simulink model "Y3Tiltrotor_sim3_INDI"  (R2025a)
settings: Solver=ode4  StartTime=0.0  StopTime=70  FixedStep=uavParam.sampleTime  RelTol=1e-3
PreLoadFcn:
  | filepath  = fileparts(get_param(bdroot, 'FileName'))
  | cd(filepath);
InitFcn:
  | Init_sim_INDI;
values from neighbouring files (symbols this model uses):
  control = struct    [Init_sim_INDI.m]
  env = struct    [InitData.m]
  flightState = struct    [Init_sim_INDI.m]
  FWSpeed0 = 15    [Init_sim_INDI.m]
  k_lpf_p = 50    [Init_sim_INDI.m]
  k_lpf_q = 80    [Init_sim_INDI.m]
  k_lpf_r = 5    [Init_sim_INDI.m]
  k_lpf_u = 10    [Init_sim_INDI.m]
  k_lpf_v = 1    [Init_sim_INDI.m]
  k_lpf_w = 50    [Init_sim_INDI.m]
  k_p = 5    [Init_sim_INDI.m]
  k_q = 20    [Init_sim_INDI.m]
  k_r = 1.5    [Init_sim_INDI.m]
  k_u = 0.5    [Init_sim_INDI.m]
  k_v = 0.5    [Init_sim_INDI.m]
  k_w = 2    [Init_sim_INDI.m]
  uavParam = struct    [InitData.m]
undefined symbols (not defined in the file or in its folder): ControlSampleTime, F, Light, MIL, Newton, Raphson
libraries: slpidlib x28, SignalEditorBlockLib x12, simulink x6, aerolibtransform2 x3, sharedtransform x3, robotcorelib x3, matrix_library x3, aerolibasang x2, aerolibutil x2, aerolibwind2 x2, shared6dof x1, aerolibatmos2 x1
(part 4 of 7)

== system Y3Tiltrotor_sim3_INDI/Subsystem/混控器/固定翼混控/固定翼模态混控 ==
  "FixedwingControlOutput " : Inport
  Action Port : ActionPort  ActionPortLabel=case [ 2 ]:
  Bus Creator : BusCreator  Inputs=2
  Bus Creator1 : BusCreator  Inputs=2
  Bus Selector : BusSelector  OutputSignals=Throttle,Tau_z,dE,dA
  Sum : Sum
  Sum1 : Sum  Inputs=+-
  toMultirotorMixer : Outport
  FixedwingCtrlSurface : Outport  Port=2
  wires:
  "FixedwingControlOutput "/1 -> Bus Selector/1
  Bus Selector/3 -> Sum1/1, Sum/1  "<dE>"
  Bus Selector/4 -> Sum1/2, Sum/2  "<dA>"
  Bus Selector/1 -> Bus Creator/1  "<Throttle>"
  Bus Creator/1 -> toMultirotorMixer/1
  Sum/1 -> Bus Creator1/1  "dA1"
  Sum1/1 -> Bus Creator1/2  "dA2"
  Bus Creator1/1 -> FixedwingCtrlSurface/1
  Bus Selector/2 -> Bus Creator/2  "<Tau_z>"

== system Y3Tiltrotor_sim3_INDI/Subsystem/混控器/固定翼混控/旋翼模态混控 ==
  Action Port : ActionPort  ActionPortLabel=case [ 0 ]:
  Bus Creator1 : BusCreator  Inputs=2
  Constant : Constant  Value=0
  Constant1 : Constant  Value=0
  FixedwingCtrlSurface : Outport
  wires:
  Constant1/1 -> Bus Creator1/2  "dA2"
  Constant/1 -> Bus Creator1/1  "dA1"
  Bus Creator1/1 -> FixedwingCtrlSurface/1

== system Y3Tiltrotor_sim3_INDI/Subsystem/混控器/多旋翼混控/Actuator To Voltage ==
  Motor Commands : Inport
  Bus Creator : BusCreator  Inputs=5
  Bus Selector : BusSelector  OutputSignals=w1,w2,w3,Tilt1,Tilt2
  Gain1 : Gain
  Gain2 : Gain
  Gain3 : Gain  Gain=1/(pi/2)
  Gain4 : Gain
  Gain5 : Gain  Gain=1/(pi/2)
  Gain6 : Gain  Commented=on  Gain=1/(uavParam.motor.RPMMAX/60)
  To PWM : Outport
  wires:
  Motor Commands/1 -> Bus Selector/1
  Bus Selector/1 -> Gain2/1  "<w1>"
  Bus Selector/3 -> Gain1/1  "<w3>"
  Bus Selector/2 -> Gain4/1  "<w2>"
  Bus Selector/4 -> Gain3/1  "<Tilt1>"
  Bus Selector/5 -> Gain5/1  "<Tilt2>"
  Gain2/1 -> Bus Creator/1  "w1"
  Gain4/1 -> Bus Creator/2  "w2"
  Gain1/1 -> Bus Creator/3  "w3"
  Gain3/1 -> Bus Creator/4  "Tilt1"
  Gain5/1 -> Bus Creator/5  "Tilt2"
  Bus Creator/1 -> To PWM/1

== system Y3Tiltrotor_sim3_INDI/Subsystem/混控器/多旋翼混控/固定翼模态混控 ==
  toMultirotorMixer : Inport
  Action Port : ActionPort  ActionPortLabel=case [ 2 ]:
  Bus Creator : BusCreator  Inputs=5
  Bus Selector : BusSelector  OutputSignals=Throttle,Tau_z
  Constant1 : Constant  Value=pi/2
  Constant2 : Constant  Value=0
  Constant7 : Constant  Value=pi/2
  Gain : Gain  Gain=1/2
  Gain1 : Gain  Gain=1/2
  Signed Sqrt : Sqrt
  Signed Sqrt1 : Sqrt
  Sum : Sum
  Sum1 : Sum  Inputs=+-
  MultirotorActuator : Outport
  wires:
  toMultirotorMixer/1 -> Bus Selector/1
  Gain/1 -> Signed Sqrt/1
  Constant1/1 -> Bus Creator/5  "Tilt2"
  Constant7/1 -> Bus Creator/4  "Tilt1"
  Gain1/1 -> Signed Sqrt1/1
  Sum1/1 -> Gain1/1
  Constant2/1 -> Bus Creator/3  "w3"
  Sum/1 -> Gain/1
  Bus Selector/1 -> Sum1/1, Sum/1  "<Throttle>"
  Bus Creator/1 -> MultirotorActuator/1
  Bus Selector/2 -> Sum/2, Sum1/2  "<Tau_z>"
  Signed Sqrt/1 -> Bus Creator/1  "w1"
  Signed Sqrt1/1 -> Bus Creator/2  "w2"

== system Y3Tiltrotor_sim3_INDI/Subsystem/混控器/多旋翼混控/旋翼模态混控 ==
  "MultirotorControlOutput " : Inport
  In Bus Element : Inport  Port=2  PortName=states  Element=Euler
  Action Port : ActionPort  ActionPortLabel=case [ 0 ]:
  Bus Creator : BusCreator  Inputs=5
  Bus Selector : BusSelector  Commented=on  OutputSignals=u_z,u_phi,u_theta
  Bus Selector1 : BusSelector  Commented=on  OutputSignals=u_x,u_psi
  Bus Selector2 : BusSelector  OutputSignals=u_z,u_phi,u_theta,u_psi,u_x
  Gain1 : Gain  Commented=on  Gain=1/(cos(asin((uavParam.motor.CQ*uavParam.geom.PropRadius)/(uavParam.motor.CT*0.24))))
  MATLAB Function : MATLAB Function  Commented=on  TreatAsAtomicUnit=on
  MATLAB Function1 : MATLAB Function  Commented=on  TreatAsAtomicUnit=on
  Multirotor Mixer1 : MATLAB Function  Commented=on  TreatAsAtomicUnit=on
  Multirotor Mixer2 (加上重力分量) : MATLAB Function  TreatAsAtomicUnit=on
  Multirotor Mixer3 : MATLAB Function  Commented=on  TreatAsAtomicUnit=on
  Multirotor Mixer4 (对应论文) : MATLAB Function  Commented=on  TreatAsAtomicUnit=on
  Saturation1 : Saturate  UpperLimit=1  LowerLimit=0
  Saturation2 : Saturate  UpperLimit=1  LowerLimit=0
  Saturation3 : Saturate  UpperLimit=1  LowerLimit=0
  Saturation4 : Saturate  UpperLimit=control.maxTiltMR  LowerLimit=control.minTiltMR
  Saturation5 : Saturate  UpperLimit=control.maxTiltMR  LowerLimit=control.minTiltMR
  Selector6 : Selector  InputPortWidth=3  IndexOptions=Index vector (dialog)  Indices=1  OutputSizes=1
  Selector7 : Selector  InputPortWidth=3  IndexOptions=Index vector (dialog)  Indices=2  OutputSizes=1
  Signed Sqrt : Sqrt
  Signed Sqrt1 : Sqrt
  Signed Sqrt2 : Sqrt
  Sin : Trigonometry  Commented=on  Operator=asin
  Sin1 : Trigonometry  Commented=on  Operator=asin
  MultirotorActuator : Outport
  wires:
  Bus Creator/1 -> MultirotorActuator/1
  MATLAB Function1/1(Tilt1) -> Sin/1
  MATLAB Function1/2(Tilt2) -> Sin1/1
  "MultirotorControlOutput "/1 -> Bus Selector/1, Bus Selector1/1, Bus Selector2/1
  Bus Selector/1 -> MATLAB Function/1(u_z)  "<u_z>"
  Bus Selector/2 -> MATLAB Function/2(u_phi)  "<u_phi>"
  Bus Selector/3 -> MATLAB Function/3(u_theta)  "<u_theta>"
  Bus Selector1/1 -> MATLAB Function1/1(u_x)  "<u_x>"
  Bus Selector1/2 -> MATLAB Function1/2(u_psi)  "<u_psi>"
  Saturation2/1 -> Bus Creator/1  "w1"
  Saturation1/1 -> Bus Creator/2  "w2"
  Saturation3/1 -> Bus Creator/3  "w3"
  Saturation4/1 -> Bus Creator/4  "Tilt1"
  Saturation5/1 -> Bus Creator/5  "Tilt2"
  Multirotor Mixer2 (加上重力分量)/4(Tilt1) -> Saturation4/1
  Multirotor Mixer2 (加上重力分量)/5(Tilt2) -> Saturation5/1
  Signed Sqrt/1 -> Saturation2/1
  Multirotor Mixer2 (加上重力分量)/1(w1) -> Signed Sqrt/1
  Multirotor Mixer2 (加上重力分量)/2(w2) -> Signed Sqrt1/1
  Signed Sqrt1/1 -> Saturation1/1
  Signed Sqrt2/1 -> Saturation3/1
  Multirotor Mixer2 (加上重力分量)/3(w3) -> Signed Sqrt2/1
  In Bus Element/1 -> Selector7/1, Selector6/1
  Selector6/1 -> [roll]
  Selector7/1 -> [pitch]
  [pitch] -> Multirotor Mixer2 (加上重力分量)/6(pitch)
  [roll] -> Multirotor Mixer2 (加上重力分量)/7(roll)
  Bus Selector2/5 -> Multirotor Mixer2 (加上重力分量)/5(u_x)  "<u_x>"
  Bus Selector2/4 -> Multirotor Mixer2 (加上重力分量)/4(u_psi)  "<u_psi>"
  Bus Selector2/3 -> Multirotor Mixer2 (加上重力分量)/3(u_theta)  "<u_theta>"
  Bus Selector2/2 -> Multirotor Mixer2 (加上重力分量)/2(u_phi)  "<u_phi>"
  Bus Selector2/1 -> Multirotor Mixer2 (加上重力分量)/1(u_z)  "<u_z>"

== system Y3Tiltrotor_sim3_INDI/Y3 Tiltrotor Aircraft Model/Subsystem/Aerodynamic Forces and Moments/Compute Air Data ==
  Vb : Inport  PortDimensions=3
  Rho : Inport  Port=2
  Bus Creator : BusCreator  Inputs=5
  Dynamic Pressure : aerolibasang/Dynamic Pressure
  "Incidence, Sideslip, & Airspeed" : aerolibasang/Incidence, Sideslip, & Airspeed
  Saturation : Saturate  UpperLimit=pi/2  LowerLimit=-pi/2
  Saturation1 : Saturate  UpperLimit=pi/2  LowerLimit=-pi/2
  Saturation2 : Saturate  UpperLimit=18.5*pi/180  LowerLimit=-13*pi/180
  Saturation3 : Saturate  UpperLimit=43*pi/180  LowerLimit=-43*pi/180
  AirData : Outport  VectorParamsAs1DForOutWhenUnconnected=off
  wires:
  Bus Creator/1 -> AirData/1
  "Incidence, Sideslip, & Airspeed"/1 -> Saturation1/1
  Rho/1 -> Dynamic Pressure/2, Bus Creator/5  "Rho"
  "Incidence, Sideslip, & Airspeed"/3 -> Bus Creator/3  "airspeed"
  Dynamic Pressure/1 -> Bus Creator/4  "q"
  Vb/1 -> "Incidence, Sideslip, & Airspeed"/1, Dynamic Pressure/1
  "Incidence, Sideslip, & Airspeed"/2 -> Saturation/1
  Saturation/1 -> Bus Creator/2  "beta"
  Saturation1/1 -> Bus Creator/1  "alpha"

== system Y3Tiltrotor_sim3_INDI/Y3 Tiltrotor Aircraft Model/Subsystem/Aerodynamic Forces and Moments/Compute Body Frame Aerodynamic Forces and Moments ==
  note: 只有力需要旋转矩阵转化，力矩不需要旋转矩阵转化。CFD拿出来的力矩数据也修正成机体坐标系下的力矩，这个模块可以最后自己搭建。
  AirData : Inport
  CtrlSurfaces : Inport  Port=2
  Aerodynamic Forces and Moment Calculations : Subsystem
  Wind frame F& M : Subsystem
  F_b : Outport  Unit=kg*m/s^2  VectorParamsAs1DForOutWhenUnconnected=off
  M_b : Outport  Port=2  Unit=kg*m/s  VectorParamsAs1DForOutWhenUnconnected=off
  wires:
  CtrlSurfaces/1 -> Wind frame F& M/2(CtrlSurfaces)
  AirData/1 -> Aerodynamic Forces and Moment Calculations/3(AirData), Wind frame F& M/1(Airdata)
  Wind frame F& M/1(coef) -> Aerodynamic Forces and Moment Calculations/1(Coef_wind)  "FM_W"
  Wind frame F& M/2(Q) -> Aerodynamic Forces and Moment Calculations/2(Q)
  Aerodynamic Forces and Moment Calculations/1(Force_b) -> F_b/1
  Aerodynamic Forces and Moment Calculations/2(Moment_b) -> M_b/1

== system Y3Tiltrotor_sim3_INDI/Y3 Tiltrotor Aircraft Model/Subsystem/Aerodynamic Forces and Moments/Compute Rho ==
  Xe : Inport
  Constant : Constant  Value=env.ISA_rho0
  Gain : Gain  Gain=-1
      settings: AttributesFormatString=Z to Alt
  Get Z : Selector  InputPortWidth=3  IndexOptions=Index vector (dialog)  Indices=[3]  OutputSizes=[(-2)]
  ISA Atmosphere Model1 : aerolibatmos2/ISA Atmosphere Model  useExtended=off  action=Warning  custom=on  viscosityOut=off  g=env.ISA_g  gamma=1.4  R=env.ISA_R  L=env.ISA_lapse  h_trop=11000  h_strat=20000  rho0=env.ISA_rho0  P0=env.ISA_P0  T0=env.ISA_T0  h0=0  S=110.4  Tref=273.15  muref=1.716e-5
  Terminator{,1..3} (4 alike) : Terminator
  Transfer Fcn : TransferFcn  Denominator=[0.01 1]
  Rho : Outport  VectorParamsAs1DForOutWhenUnconnected=off
  wires:
  ISA Atmosphere Model1/2 -> Terminator1/1
  ISA Atmosphere Model1/1 -> Terminator/1  "OAT"
  Gain/1 -> ISA Atmosphere Model1/1
  Get Z/1 -> Transfer Fcn/1
  Transfer Fcn/1 -> Gain/1
  ISA Atmosphere Model1/3 -> Terminator2/1  "static"
  Xe/1 -> Get Z/1
  Constant/1 -> Rho/1
  ISA Atmosphere Model1/4 -> Terminator3/1

== system Y3Tiltrotor_sim3_INDI/Y3 Tiltrotor Aircraft Model/Subsystem/GroundModel1/Ground Model New ==
  note: z=Xe(3)-terrainZ;
      | if z>=0
      |
      |     if z<0.05
      |          F1(3)=-mg(3)-10*Ve(3);
      |     elseif z<0.1
      |         F1(3)=-mg(3)-0.5*z-20*Ve(3);
      |     else
      |          F1(3)=-mg(3)-1*z-50*Ve(3);
      |     end
      |
      |
      |     F1(1)=-2*Ve(1);
      |     F1(2)=-50*Ve(2);
      |     M1=-20*[Quet(2);Quet(3);Quet(4)]-5*wb;
      |     M1 = M1 * abs(mg(3))*0.0333;
      | end
  mg : Inport  PortDimensions=3
  wb : Inport  Port=2  PortDimensions=3
  Xe : Inport  Port=3  PortDimensions=3
  Ve : Inport  Port=4
  Quet : Inport  Port=5  PortDimensions=4
  TerrainZ : Inport  Port=6
  Abs : Abs  SaturateOnIntegerOverflow=off
  Constant : Constant  Value=0
  Demux : Demux  Outputs=3
  F0M0 : Constant  Value=[0,0,0]
  F0M1 : Constant  Value=[0,0,0]
  Gain : Gain  Gain=-0.1
  Gain1 : Gain  Gain=-1
  Gain2 : Gain  Gain=-5
  Gain3 : Gain  Gain=-20
  Gain4 : Gain  Gain=0.0333
  If : If  IfExpression=u1 < 0.05  ElseIfExpressions=u1<0.1
  If Action Subsystem : Subsystem  TreatAsAtomicUnit=on
  If Action Subsystem1 : Subsystem  TreatAsAtomicUnit=on
  If Action Subsystem2 : Subsystem  TreatAsAtomicUnit=on
  Merge : Merge  Inputs=3  InitialOutput=0
  Mux : Mux  Inputs=3
  Product : Product
  Selector : Selector  InputPortWidth=3  IndexOptions=Index vector (dialog)  Indices=[3]  OutputSizes=1
  Selector1 : Selector  InputPortWidth=3  IndexOptions=Index vector (dialog)  Indices=[3]  OutputSizes=1
  Selector2 : Selector  InputPortWidth=4  IndexOptions=Index vector (dialog)  Indices=[2:4]  OutputSizes=1
  Sum : Sum  Inputs=|+-
  Sum1 : Sum  Inputs=|++
  Switch : Switch  SaturateOnIntegerOverflow=off  InputSameDT=off
  Switch1 : Switch  SaturateOnIntegerOverflow=off  InputSameDT=off
  F1 : Outport  VectorParamsAs1DForOutWhenUnconnected=off
  M1 : Outport  Port=2  VectorParamsAs1DForOutWhenUnconnected=off
  wires:
  Gain2/1 -> Sum1/2
  Merge/1 -> Mux/3  "F13"
  Switch1/1 -> F1/1
  Abs/1 -> Gain4/1
  Selector2/1 -> Gain3/1
  F0M0/1 -> Switch1/3, Switch/3
  Demux/1 -> Gain/1  "ve1"
  If Action Subsystem1/1(F13) -> Merge/2
  Quet/1 -> Selector2/1
  Ve/1 -> Demux/1
  Mux/1 -> Switch1/1  "F1"
  Gain3/1 -> Sum1/1
  Switch/1 -> M1/1
  Sum1/1 -> Product/1
  Gain4/1 -> Product/2
  Xe/1 -> Selector/1
  Demux/3 -> If Action Subsystem1/2(ve3), If Action Subsystem2/2(ve3), If Action Subsystem/2(ve3)  "ve3"
  Selector/1 -> Sum/1
  mg/1 -> Selector1/1
  wb/1 -> Gain2/1
  TerrainZ/1 -> Sum/2
  Sum/1 -> Switch1/2, Switch/2, If Action Subsystem2/3(z), If Action Subsystem1/3(z), If/1  "Z"
  If/1 -> If Action Subsystem/Action
  If Action Subsystem2/1(F13) -> Merge/3
  If Action Subsystem/1(F13) -> Merge/1
  If/3 -> If Action Subsystem2/Action
  If/2 -> If Action Subsystem1/Action
  Selector1/1 -> If Action Subsystem/1(mg3), Abs/1, If Action Subsystem2/1(mg3), If Action Subsystem1/1(mg3)
  Demux/2 -> Gain1/1  "ve2"
  Gain/1 -> Mux/1  "F11"
  Gain1/1 -> Mux/2  "F12"
  F0M1/1 -> Switch/1

== system Y3Tiltrotor_sim3_INDI/Y3 Tiltrotor Aircraft Model/Subsystem/GroundModel1/OnGroundFaceup ==
  Eular(rad) : Inport
  ModelInit_GroundSlope : Constant  Value=[0,0]
  Mux : Mux  Inputs=2
  Selector : Selector  InputPortWidth=3  IndexOptions=Index vector (dialog)  Indices=[3]  OutputSizes=1
  y : Outport  VectorParamsAs1DForOutWhenUnconnected=off
  wires:
  Mux/1 -> y/1
  ModelInit_GroundSlope/1 -> Mux/1
  Selector/1 -> Mux/2
  Eular(rad)/1 -> Selector/1

== system Y3Tiltrotor_sim3_INDI/Y3 Tiltrotor Aircraft Model/Subsystem/Propulsion/Rotor Assembly 1 ==
  N : Inport
  Arm : Inport  Port=2
  Tilt : Inport  Port=3
  TurnDirection : Inport  Port=4
  Rho : Inport  Port=5
  Add1 : Sum
  Adjust Force to Body Frame : Subsystem
  Cross Product1 : matrix_library/Cross Product
  Gain : Gain  Gain=2*pi
  Gain1 : Gain  Gain=uavParam.motor.RPMMAX/60
  Product1 : Product
  Rotor : Rotor  CT=uavParam.motor.CT  CQ=uavParam.motor.CQ  radius=uavParam.geom.PropRadius
      settings: LibrarySourceBlock=aerolibrotor/Rotor
  Saturation : Saturate  UpperLimit=1  LowerLimit=0
  F : Outport
  M : Outport  Port=2
  w : Outport  Port=3
  wires:
  TurnDirection/1 -> Adjust Force to Body Frame/3(TurnDirection), Product1/1
  Adjust Force to Body Frame/1(Fbody) -> F/1, Cross Product1/2  "F_rotor1"
  Product1/1 -> Add1/2
  Cross Product1/1 -> Add1/1
  Arm/1 -> Cross Product1/1
  Rho/1 -> Rotor/2  "Rho"
  Add1/1 -> M/1  "M_rotor1"
  Rotor/2 -> Product1/2  "M_1"
  Saturation/1 -> Gain1/1
  N/1 -> Saturation/1
  Gain1/1 -> Gain/1, w/1  "W"
  Tilt/1 -> Adjust Force to Body Frame/2(Tilt)
  Rotor/1 -> Adjust Force to Body Frame/1(Fmotor)  "T_1"
  Gain/1 -> Rotor/1

== system Y3Tiltrotor_sim3_INDI/Y3 Tiltrotor Aircraft Model/Subsystem/Propulsion/Rotor Assembly 2 ==
  N : Inport
  Arm : Inport  Port=2
  Tilt : Inport  Port=3
  TurnDirection : Inport  Port=4
  Rho : Inport  Port=5
  Add1 : Sum
  Adjust Force to Body Frame : Subsystem
  Cross Product1 : matrix_library/Cross Product
  Gain : Gain  Gain=2*pi
  Gain1 : Gain  Gain=uavParam.motor.RPMMAX/60
  Product1 : Product
  Rotor1 : Rotor  CT=uavParam.motor.CT  CQ=uavParam.motor.CQ  radius=uavParam.geom.PropRadius
      settings: LibrarySourceBlock=aerolibrotor/Rotor
  Saturation1 : Saturate  UpperLimit=1  LowerLimit=0
  F : Outport
  M : Outport  Port=2
  w : Outport  Port=3
  wires:
  Gain1/1 -> Gain/1, w/1  "W"
  N/1 -> Saturation1/1
  Saturation1/1 -> Gain1/1
  Gain/1 -> Rotor1/1
  Rotor1/2 -> Product1/2
  Add1/1 -> M/1
  Rho/1 -> Rotor1/2
  Arm/1 -> Cross Product1/1
  Cross Product1/1 -> Add1/1
  Product1/1 -> Add1/2
  Adjust Force to Body Frame/1(Fbody) -> F/1, Cross Product1/2
  TurnDirection/1 -> Product1/1, Adjust Force to Body Frame/3(TurnDirection)
  Tilt/1 -> Adjust Force to Body Frame/2(Tilt)
  Rotor1/1 -> Adjust Force to Body Frame/1(Fmotor)

== system Y3Tiltrotor_sim3_INDI/Y3 Tiltrotor Aircraft Model/Subsystem/Propulsion/Rotor Assembly 3  ==
  note: 需要测出电机螺旋桨的Ct和Cq，看尾电机的安装角在理论上是否能够抵消电机自身的反扭力矩。
  note: 从后侧看，尾电机并没有垂直安装，具有向左倾斜的初始安装角，主要用于抵消尾电机的反扭矩，量角器测量初始安装角大约倾斜了10度。
  N : Inport
  Arm : Inport  Port=2
  Tilt : Inport  Port=3
  TurnDirection : Inport  Port=4
  Rho : Inport  Port=5
  Add1 : Sum
  Adjust Force to Body Frame : Subsystem
  Cross Product1 : matrix_library/Cross Product
  Gain : Gain  Gain=2*pi
  Gain1 : Gain  Gain=uavParam.motor.RPMMAX/60
  Gain2 : Gain  Gain=0
  Product1 : Product
  Rotor1 : Rotor  CT=uavParam.motor.CT  CQ=uavParam.motor.CQ  radius=uavParam.geom.PropRadius
      settings: LibrarySourceBlock=aerolibrotor/Rotor
  Saturation1 : Saturate  UpperLimit=1  LowerLimit=0
  F : Outport
  M : Outport  Port=2
  w : Outport  Port=3
  wires:
  TurnDirection/1 -> Adjust Force to Body Frame/3(TurnDirection), Product1/1
  Adjust Force to Body Frame/1(Fbody) -> Cross Product1/2, F/1
  Product1/1 -> Add1/2
  Cross Product1/1 -> Add1/1
  Arm/1 -> Cross Product1/1
  Rho/1 -> Rotor1/2
  Add1/1 -> M/1
  Rotor1/2 -> Gain2/1
  Gain/1 -> Rotor1/1
  Saturation1/1 -> Gain1/1
  N/1 -> Saturation1/1
  Gain1/1 -> w/1, Gain/1  "W"
  Tilt/1 -> Adjust Force to Body Frame/2(Tilt)
  Rotor1/1 -> Adjust Force to Body Frame/1(Fmotor)
  Gain2/1 -> Product1/2

== system Y3Tiltrotor_sim3_INDI/Y3 Tiltrotor Aircraft Model/Subsystem/Propulsion/Tilt Servo Dynamics ==
  TiltA : Inport
  TiltB : Inport  Port=2
  Gain : Gain  Gain=180/pi
  Gain1 : Gain  Gain=180/pi
  Gain2 : Gain  Gain=pi/2
  Gain3 : Gain  Gain=pi/2
  IC2 : InitialCondition  Commented=on  Value=0
  Servo Dynamics2 : TransferFcn  Commented=on  Denominator=[0.1 1]
  Terminator : Terminator
  Terminator1 : Terminator
  Tilt1 : Outport
  Tilt2 : Outport  Port=2
  wires:
  TiltB/1 -> Gain3/1
  Gain3/1 -> Gain1/1, Tilt2/1  "Tilt2"
  Gain2/1 -> Tilt1/1, Gain/1  "Tilt1"
  TiltA/1 -> Gain2/1
  Servo Dynamics2/1 -> IC2/1
  Gain/1 -> Terminator/1  "Tilt1_deg"
  Gain1/1 -> Terminator1/1  "Tilt2_deg"

== system Y3Tiltrotor_sim3_INDI/Y3 Tiltrotor Aircraft Model/Subsystem/Weather Model_org/ Compute Norm ==
  <Ve> : Inport
  Dot Product : DotProduct  OutDataTypeStr=Inherit: Inherit via internal rule
  Math Function1 : Sqrt  AlgorithmType=Newton-Raphson
      settings: AttributesFormatString=%<AlgorithmType>
  Zero Bound : Saturate  UpperLimit=inf  LowerLimit=0.001
      settings: AttributesFormatString="[%<LowerLimit>  %<UpperLimit>]"
  V : Outport  VectorParamsAs1DForOutWhenUnconnected=off
  wires:
  Dot Product/1 -> Zero Bound/1
  Zero Bound/1 -> Math Function1/1
  <Ve>/1 -> Dot Product/2, Dot Product/1
  Math Function1/1 -> V/1

== system Y3Tiltrotor_sim3_INDI/Y3 Tiltrotor Aircraft Model/Subsystem/Weather Model_org/RL2B ==
  Euler : Inport
  Rotation Angles to Direction Cosine Matrix : sharedtransform/Rotation Angles to Direction Cosine Matrix  rotationOrder=ZYX  aMode=aMode
  Selector : Selector  InputPortWidth=3  IndexOptions=Index vector (dialog)  Indices=[3 2 1]  OutputSizes=1
  RL2B : Outport  VectorParamsAs1DForOutWhenUnconnected=off
  wires:
  Rotation Angles to Direction Cosine Matrix/1 -> RL2B/1
  Euler/1 -> Selector/1
  Selector/1 -> Rotation Angles to Direction Cosine Matrix/1

== system Y3Tiltrotor_sim3_INDI/Y3 Tiltrotor Aircraft Model/Subsystem/Weather Model_org/[0, pi] Wrap Around ==
  Euler : Inport
  Compare To Zero : simulink/Logic and Bit Operations/Compare To Zero  relop=>=  OutDataTypeStr=uint8  ZeroCross=off
  Logical Operator : Logic  Operator=NOT  AllPortsSameDT=off  OutDataTypeStr=boolean
  Merge : Merge  InitialOutput=0
  Mux2 : Mux  Inputs=2
  Negative Yaw : Subsystem
  Positive Yaw : Subsystem
  Selector1 : Selector  InputPortWidth=3  IndexOptions=Index vector (dialog)  Indices=[1 2]  OutputSizes=1
  Selector2 : Selector  InputPortWidth=3  IndexOptions=Index vector (dialog)  Indices=[3]  OutputSizes=1
  Wrapped : Outport  VectorParamsAs1DForOutWhenUnconnected=off
  wires:
  Negative Yaw/1(yaw_wr) -> Merge/2
  Positive Yaw/1(yaw_wr) -> Merge/1
  Merge/1 -> Mux2/2
  Logical Operator/1 -> Negative Yaw/Enable
  Compare To Zero/1 -> Logical Operator/1, Positive Yaw/Enable
  Selector2/1 -> Negative Yaw/1(yaw), Positive Yaw/1(yaw), Compare To Zero/1
  Mux2/1 -> Wrapped/1
  Selector1/1 -> Mux2/1
  Euler/1 -> Selector1/1, Selector2/1

== system Y3Tiltrotor_sim3_INDI/Subsystem/固定翼模态/高度-速度控制/定速模式/Subsystem1 ==
  Manual : Inport
  Ve : Inport  Port=2
  Height_d : Inport  Port=3
  Manual Vz_d : Inport  Port=4
  Xe : Inport  Port=5
  PID Controller1 : slpidlib/PID Controller  Controller=PID  Form=Parallel  TimeDomain=Continuous-time  UseExternalTs=off  SampleTime=ControlSampleTime  IntegratorMethod=Forward Euler  FilterMethod=Forward Euler  ControllerParametersSource=internal  P=control.FW.vz_P  I=control.FW.vz_I  UseKiTs=off  D=control.FW.vz_D  UseExternalDerivativeSource=off  N=100  UseFilter=on  TunerSelectOption=Transfer Function Based (PID Tuner App)  InitialConditionSource=internal  InitialConditionForIntegrator=0  InitialConditionForFilter=0  DifferentiatorICPrevScaledInput=0  ExternalReset=none  TrackingMode=off  Kt=1  LimitOutput=on  SatLimitsSource=internal  UpperSaturationLimit=control.maxPitch  LowerSaturationLimit=control.minPitch  LinearizeAsGain=on  AntiWindupMode=clamping  Kb=1  LimitIntegrator=off  UpperIntegratorSaturationLimit=inf  LowerIntegratorSaturationLimit=-inf  POutMin=[]  POutMax=[]  IOutMin=[]  IOutMax=[]  DOutMin=[]  DOutMax=[]  NOutMin=[]  NOutMax=[]  SumOutMin=[]  SumOutMax=[]  SaturationOutMin=[]  SaturationOutMax=[]  PParamMin=[]  PParamMax=[]  IParamMin=[]  IParamMax=[]  DParamMin=[]  DParamMax=[]  NParamMin=[]  NParamMax=[]  KbParamMin=[]  KbParamMax=[]  KtParamMin=[]  KtParamMax=[]  KbOutMin=[]  KbOutMax=[]  KtOutMin=[]  KtOutMax=[]  IntegratorOutMin=[]  IntegratorOutMax=[]  FilterOutMin=[]  FilterOutMax=[]  SumI1OutMin=[]  SumI1OutMax=[]  SumI2OutMin=[]  SumI2OutMax=[]  SumI3OutMin=[]  SumI3OutMax=[]  SumI4OutMin=[]  SumI4OutMax=[]  SumDOutMin=[]  SumDOutMax=[]  DifferentiatorOutMin=[]  DifferentiatorOutMax=[]  FilterDiffOutCoefMin=[]  FilterDiffOutCoefMax=[]  ReciprocalOutMin=[]  ReciprocalOutMax=[]  SumDenOutMin=[]  SumDenOutMax=[]  SumNumOutMin=[]  SumNumOutMax=[]  DivideOutMin=[]  DivideOutMax=[]  UdiffTsProdOutMin=[]  UdiffTsProdOutMax=[]  NTsProdOutMin=[]  NTsProdOutMax=[]  UintegralTsProdOutMin=[]  UintegralTsProdOutMax=[]  UngainTsProdOutMin=[]  UngainTsProdOutMax=[]  ClampingZeroOutDataTypeStr=Inherit: Inherit via back propagation  ClampingZeroOutMin=[]  ClampingZeroOutMax=[]  FilterDenConstantOutDataTypeStr=Inherit: Inherit via back propagation  FilterDenConstantOutMin=[]  FilterDenConstantOutMax=[]  PCopyOutDataTypeStr=Inherit: Inherit via back propagation  PCopyOutMin=[]  PCopyOutMax=[]  NCopyOutDataTypeStr=Inherit: Inherit via back propagation  NCopyOutMin=[]  NCopyOutMax=[]  IntegratorContinuousStateAttributes=''  IntegratorStateMustResolveToSignalObject=off  IntegratorRTWStateStorageClass=Auto  FilterContinuousStateAttributes=''  FilterStateMustResolveToSignalObject=off  FilterRTWStateStorageClass=Auto  ParallelPVariant=InternalParameters  IdealPVariant=Disabled  IVariant=InternalParameters  DVariant=InternalParameters  IntegratorVariant=Continuous  SatVariant=Enabled  AWVariant=ContClampingParallel  PCopyVariant=Disabled  TRVariant=Disabled  FdbkBlocksVariant=Forward  IdealPFdbkVariant=Disabled  SatFdbkVariant=Disabled  DerivativeFilterVariant=ContFilter  NVariant=InternalParameters  NCopyVariant=Disabled  FilterICVariant=InternalICsFilter  IntegratorICVariant=InternalICs  ExternalResetVariant=Disabled  TRSumVariant=Passthrough  SumFdbkVariant=Disabled  SumVariant=Sum_PID  TsampFilterVariant=InternalTs  TsampNgainVariant=Passthrough  TsampIntegralVariant=Disabled_SignalSpec  ExternalSaturationOutDataTypeStr=Inherit: Same as second input  DerivativeSourceVariant=ErrorSignal  PreIntVariant=InternalPreInt
  Selector1 : Selector  InputPortWidth=3  IndexOptions=Index vector (dialog)  Indices=3  OutputSizes=1
  Subsystem : Subsystem
  Sum1 : Sum  Inputs=|+-
  Transfer Fcn : TransferFcn  Numerator=[5]  Denominator=[1 5]
  Unary Minus1 : UnaryMinus
  Pitch_d_alt : Outport
  wires:
  Ve/1 -> Selector1/1
  Unary Minus1/1 -> Sum1/2
  Subsystem/1(Vz_d) -> Transfer Fcn/1
  Sum1/1 -> PID Controller1/1
  Selector1/1 -> Unary Minus1/1
  Transfer Fcn/1 -> Sum1/1
  Manual/1 -> Subsystem/1(Manual)
  Height_d/1 -> Subsystem/2(Height_d)
  Manual Vz_d/1 -> Subsystem/3(Manual Vz_d)
  PID Controller1/1 -> Pitch_d_alt/1
  Xe/1 -> Subsystem/4(Xe)

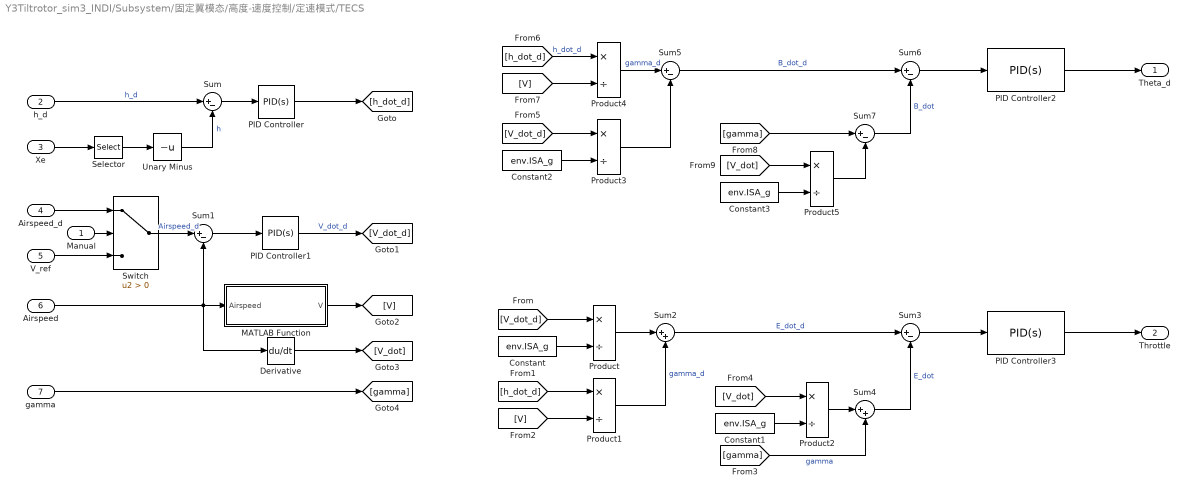
== system Y3Tiltrotor_sim3_INDI/Subsystem/固定翼模态/高度-速度控制/定速模式/TECS ==
  Manual : Inport
  h_d : Inport  Port=2
  Xe : Inport  Port=3
  Airspeed_d : Inport  Port=4
  V_ref : Inport  Port=5
  Airspeed : Inport  Port=6
  gamma : Inport  Port=7
  Constant{,1..3} (4 alike) : Constant  Value=env.ISA_g
  Derivative : Derivative
  MATLAB Function : MATLAB Function  TreatAsAtomicUnit=on
  PID Controller : slpidlib/PID Controller  Controller=PID  Form=Parallel  TimeDomain=Continuous-time  UseExternalTs=off  SampleTime=ControlSampleTime  IntegratorMethod=Forward Euler  FilterMethod=Forward Euler  ControllerParametersSource=internal  P=control.FW.TECSalt_P  I=control.FW.TECSalt_I  UseKiTs=off  D=control.FW.TECSalt_D  UseExternalDerivativeSource=off  N=100  UseFilter=on  TunerSelectOption=Transfer Function Based (PID Tuner App)  InitialConditionSource=internal  InitialConditionForIntegrator=0  InitialConditionForFilter=0  DifferentiatorICPrevScaledInput=0  ExternalReset=none  TrackingMode=off  Kt=1  LimitOutput=on  SatLimitsSource=internal  UpperSaturationLimit=control.maxClimbRate  LowerSaturationLimit=control.maxDescendRate  LinearizeAsGain=on  AntiWindupMode=clamping  Kb=1  LimitIntegrator=off  UpperIntegratorSaturationLimit=inf  LowerIntegratorSaturationLimit=-inf  POutMin=[]  POutMax=[]  IOutMin=[]  IOutMax=[]  DOutMin=[]  DOutMax=[]  NOutMin=[]  NOutMax=[]  SumOutMin=[]  SumOutMax=[]  SaturationOutMin=[]  SaturationOutMax=[]  PParamMin=[]  PParamMax=[]  IParamMin=[]  IParamMax=[]  DParamMin=[]  DParamMax=[]  NParamMin=[]  NParamMax=[]  KbParamMin=[]  KbParamMax=[]  KtParamMin=[]  KtParamMax=[]  KbOutMin=[]  KbOutMax=[]  KtOutMin=[]  KtOutMax=[]  IntegratorOutMin=[]  IntegratorOutMax=[]  FilterOutMin=[]  FilterOutMax=[]  SumI1OutMin=[]  SumI1OutMax=[]  SumI2OutMin=[]  SumI2OutMax=[]  SumI3OutMin=[]  SumI3OutMax=[]  SumI4OutMin=[]  SumI4OutMax=[]  SumDOutMin=[]  SumDOutMax=[]  DifferentiatorOutMin=[]  DifferentiatorOutMax=[]  FilterDiffOutCoefMin=[]  FilterDiffOutCoefMax=[]  ReciprocalOutMin=[]  ReciprocalOutMax=[]  SumDenOutMin=[]  SumDenOutMax=[]  SumNumOutMin=[]  SumNumOutMax=[]  DivideOutMin=[]  DivideOutMax=[]  UdiffTsProdOutMin=[]  UdiffTsProdOutMax=[]  NTsProdOutMin=[]  NTsProdOutMax=[]  UintegralTsProdOutMin=[]  UintegralTsProdOutMax=[]  UngainTsProdOutMin=[]  UngainTsProdOutMax=[]  ClampingZeroOutDataTypeStr=Inherit: Inherit via back propagation  ClampingZeroOutMin=[]  ClampingZeroOutMax=[]  FilterDenConstantOutDataTypeStr=Inherit: Inherit via back propagation  FilterDenConstantOutMin=[]  FilterDenConstantOutMax=[]  PCopyOutDataTypeStr=Inherit: Inherit via back propagation  PCopyOutMin=[]  PCopyOutMax=[]  NCopyOutDataTypeStr=Inherit: Inherit via back propagation  NCopyOutMin=[]  NCopyOutMax=[]  IntegratorContinuousStateAttributes=''  IntegratorStateMustResolveToSignalObject=off  IntegratorRTWStateStorageClass=Auto  FilterContinuousStateAttributes=''  FilterStateMustResolveToSignalObject=off  FilterRTWStateStorageClass=Auto  ParallelPVariant=InternalParameters  IdealPVariant=Disabled  IVariant=InternalParameters  DVariant=InternalParameters  IntegratorVariant=Continuous  SatVariant=Enabled  AWVariant=ContClampingParallel  PCopyVariant=Disabled  TRVariant=Disabled  FdbkBlocksVariant=Forward  IdealPFdbkVariant=Disabled  SatFdbkVariant=Disabled  DerivativeFilterVariant=ContFilter  NVariant=InternalParameters  NCopyVariant=Disabled  FilterICVariant=InternalICsFilter  IntegratorICVariant=InternalICs  ExternalResetVariant=Disabled  TRSumVariant=Passthrough  SumFdbkVariant=Disabled  SumVariant=Sum_PID  TsampFilterVariant=InternalTs  TsampNgainVariant=Passthrough  TsampIntegralVariant=Disabled_SignalSpec  ExternalSaturationOutDataTypeStr=Inherit: Same as second input  DerivativeSourceVariant=ErrorSignal  PreIntVariant=InternalPreInt
  PID Controller1 : slpidlib/PID Controller  Controller=PID  Form=Parallel  TimeDomain=Continuous-time  UseExternalTs=off  SampleTime=ControlSampleTime  IntegratorMethod=Forward Euler  FilterMethod=Forward Euler  ControllerParametersSource=internal  P=control.FW.TECSairspeed_P  I=control.FW.TECSairspeed_I  UseKiTs=off  D=control.FW.TECSairspeed_D  UseExternalDerivativeSource=off  N=100  UseFilter=on  TunerSelectOption=Transfer Function Based (PID Tuner App)  InitialConditionSource=internal  InitialConditionForIntegrator=0  InitialConditionForFilter=0  DifferentiatorICPrevScaledInput=0  ExternalReset=none  TrackingMode=off  Kt=1  LimitOutput=on  SatLimitsSource=internal  UpperSaturationLimit=100  LowerSaturationLimit=-100  LinearizeAsGain=on  AntiWindupMode=clamping  Kb=1  LimitIntegrator=off  UpperIntegratorSaturationLimit=inf  LowerIntegratorSaturationLimit=-inf  POutMin=[]  POutMax=[]  IOutMin=[]  IOutMax=[]  DOutMin=[]  DOutMax=[]  NOutMin=[]  NOutMax=[]  SumOutMin=[]  SumOutMax=[]  SaturationOutMin=[]  SaturationOutMax=[]  PParamMin=[]  PParamMax=[]  IParamMin=[]  IParamMax=[]  DParamMin=[]  DParamMax=[]  NParamMin=[]  NParamMax=[]  KbParamMin=[]  KbParamMax=[]  KtParamMin=[]  KtParamMax=[]  KbOutMin=[]  KbOutMax=[]  KtOutMin=[]  KtOutMax=[]  IntegratorOutMin=[]  IntegratorOutMax=[]  FilterOutMin=[]  FilterOutMax=[]  SumI1OutMin=[]  SumI1OutMax=[]  SumI2OutMin=[]  SumI2OutMax=[]  SumI3OutMin=[]  SumI3OutMax=[]  SumI4OutMin=[]  SumI4OutMax=[]  SumDOutMin=[]  SumDOutMax=[]  DifferentiatorOutMin=[]  DifferentiatorOutMax=[]  FilterDiffOutCoefMin=[]  FilterDiffOutCoefMax=[]  ReciprocalOutMin=[]  ReciprocalOutMax=[]  SumDenOutMin=[]  SumDenOutMax=[]  SumNumOutMin=[]  SumNumOutMax=[]  DivideOutMin=[]  DivideOutMax=[]  UdiffTsProdOutMin=[]  UdiffTsProdOutMax=[]  NTsProdOutMin=[]  NTsProdOutMax=[]  UintegralTsProdOutMin=[]  UintegralTsProdOutMax=[]  UngainTsProdOutMin=[]  UngainTsProdOutMax=[]  ClampingZeroOutDataTypeStr=Inherit: Inherit via back propagation  ClampingZeroOutMin=[]  ClampingZeroOutMax=[]  FilterDenConstantOutDataTypeStr=Inherit: Inherit via back propagation  FilterDenConstantOutMin=[]  FilterDenConstantOutMax=[]  PCopyOutDataTypeStr=Inherit: Inherit via back propagation  PCopyOutMin=[]  PCopyOutMax=[]  NCopyOutDataTypeStr=Inherit: Inherit via back propagation  NCopyOutMin=[]  NCopyOutMax=[]  IntegratorContinuousStateAttributes=''  IntegratorStateMustResolveToSignalObject=off  IntegratorRTWStateStorageClass=Auto  FilterContinuousStateAttributes=''  FilterStateMustResolveToSignalObject=off  FilterRTWStateStorageClass=Auto  ParallelPVariant=InternalParameters  IdealPVariant=Disabled  IVariant=InternalParameters  DVariant=InternalParameters  IntegratorVariant=Continuous  SatVariant=Enabled  AWVariant=ContClampingParallel  PCopyVariant=Disabled  TRVariant=Disabled  FdbkBlocksVariant=Forward  IdealPFdbkVariant=Disabled  SatFdbkVariant=Disabled  DerivativeFilterVariant=ContFilter  NVariant=InternalParameters  NCopyVariant=Disabled  FilterICVariant=InternalICsFilter  IntegratorICVariant=InternalICs  ExternalResetVariant=Disabled  TRSumVariant=Passthrough  SumFdbkVariant=Disabled  SumVariant=Sum_PID  TsampFilterVariant=InternalTs  TsampNgainVariant=Passthrough  TsampIntegralVariant=Disabled_SignalSpec  ExternalSaturationOutDataTypeStr=Inherit: Same as second input  DerivativeSourceVariant=ErrorSignal  PreIntVariant=InternalPreInt
  PID Controller2 : slpidlib/PID Controller  Controller=PID  Form=Parallel  TimeDomain=Continuous-time  UseExternalTs=off  SampleTime=ControlSampleTime  IntegratorMethod=Forward Euler  FilterMethod=Forward Euler  ControllerParametersSource=internal  P=control.FW.B_P  I=control.FW.B_I  UseKiTs=off  D=control.FW.B_D  UseExternalDerivativeSource=off  N=100  UseFilter=on  TunerSelectOption=Transfer Function Based (PID Tuner App)  InitialConditionSource=internal  InitialConditionForIntegrator=0  InitialConditionForFilter=0  DifferentiatorICPrevScaledInput=0  ExternalReset=none  TrackingMode=off  Kt=1  LimitOutput=on  SatLimitsSource=internal  UpperSaturationLimit=control.FWmaxPitch  LowerSaturationLimit=control.FWminPitch  LinearizeAsGain=on  AntiWindupMode=clamping  Kb=1  LimitIntegrator=off  UpperIntegratorSaturationLimit=inf  LowerIntegratorSaturationLimit=-inf  POutMin=[]  POutMax=[]  IOutMin=[]  IOutMax=[]  DOutMin=[]  DOutMax=[]  NOutMin=[]  NOutMax=[]  SumOutMin=[]  SumOutMax=[]  SaturationOutMin=[]  SaturationOutMax=[]  PParamMin=[]  PParamMax=[]  IParamMin=[]  IParamMax=[]  DParamMin=[]  DParamMax=[]  NParamMin=[]  NParamMax=[]  KbParamMin=[]  KbParamMax=[]  KtParamMin=[]  KtParamMax=[]  KbOutMin=[]  KbOutMax=[]  KtOutMin=[]  KtOutMax=[]  IntegratorOutMin=[]  IntegratorOutMax=[]  FilterOutMin=[]  FilterOutMax=[]  SumI1OutMin=[]  SumI1OutMax=[]  SumI2OutMin=[]  SumI2OutMax=[]  SumI3OutMin=[]  SumI3OutMax=[]  SumI4OutMin=[]  SumI4OutMax=[]  SumDOutMin=[]  SumDOutMax=[]  DifferentiatorOutMin=[]  DifferentiatorOutMax=[]  FilterDiffOutCoefMin=[]  FilterDiffOutCoefMax=[]  ReciprocalOutMin=[]  ReciprocalOutMax=[]  SumDenOutMin=[]  SumDenOutMax=[]  SumNumOutMin=[]  SumNumOutMax=[]  DivideOutMin=[]  DivideOutMax=[]  UdiffTsProdOutMin=[]  UdiffTsProdOutMax=[]  NTsProdOutMin=[]  NTsProdOutMax=[]  UintegralTsProdOutMin=[]  UintegralTsProdOutMax=[]  UngainTsProdOutMin=[]  UngainTsProdOutMax=[]  ClampingZeroOutDataTypeStr=Inherit: Inherit via back propagation  ClampingZeroOutMin=[]  ClampingZeroOutMax=[]  FilterDenConstantOutDataTypeStr=Inherit: Inherit via back propagation  FilterDenConstantOutMin=[]  FilterDenConstantOutMax=[]  PCopyOutDataTypeStr=Inherit: Inherit via back propagation  PCopyOutMin=[]  PCopyOutMax=[]  NCopyOutDataTypeStr=Inherit: Inherit via back propagation  NCopyOutMin=[]  NCopyOutMax=[]  IntegratorContinuousStateAttributes=''  IntegratorStateMustResolveToSignalObject=off  IntegratorRTWStateStorageClass=Auto  FilterContinuousStateAttributes=''  FilterStateMustResolveToSignalObject=off  FilterRTWStateStorageClass=Auto  ParallelPVariant=InternalParameters  IdealPVariant=Disabled  IVariant=InternalParameters  DVariant=InternalParameters  IntegratorVariant=Continuous  SatVariant=Enabled  AWVariant=ContClampingParallel  PCopyVariant=Disabled  TRVariant=Disabled  FdbkBlocksVariant=Forward  IdealPFdbkVariant=Disabled  SatFdbkVariant=Disabled  DerivativeFilterVariant=ContFilter  NVariant=InternalParameters  NCopyVariant=Disabled  FilterICVariant=InternalICsFilter  IntegratorICVariant=InternalICs  ExternalResetVariant=Disabled  TRSumVariant=Passthrough  SumFdbkVariant=Disabled  SumVariant=Sum_PID  TsampFilterVariant=InternalTs  TsampNgainVariant=Passthrough  TsampIntegralVariant=Disabled_SignalSpec  ExternalSaturationOutDataTypeStr=Inherit: Same as second input  DerivativeSourceVariant=ErrorSignal  PreIntVariant=InternalPreInt
  PID Controller3 : slpidlib/PID Controller  Controller=PID  Form=Parallel  TimeDomain=Continuous-time  UseExternalTs=off  SampleTime=ControlSampleTime  IntegratorMethod=Forward Euler  FilterMethod=Forward Euler  ControllerParametersSource=internal  P=control.FW.E_P  I=control.FW.E_I  UseKiTs=off  D=control.FW.E_D  UseExternalDerivativeSource=off  N=100  UseFilter=on  TunerSelectOption=Transfer Function Based (PID Tuner App)  InitialConditionSource=internal  InitialConditionForIntegrator=0  InitialConditionForFilter=0  DifferentiatorICPrevScaledInput=0  ExternalReset=none  TrackingMode=off  Kt=1  LimitOutput=on  SatLimitsSource=internal  UpperSaturationLimit=1  LowerSaturationLimit=0  LinearizeAsGain=on  AntiWindupMode=clamping  Kb=1  LimitIntegrator=off  UpperIntegratorSaturationLimit=inf  LowerIntegratorSaturationLimit=-inf  POutMin=[]  POutMax=[]  IOutMin=[]  IOutMax=[]  DOutMin=[]  DOutMax=[]  NOutMin=[]  NOutMax=[]  SumOutMin=[]  SumOutMax=[]  SaturationOutMin=[]  SaturationOutMax=[]  PParamMin=[]  PParamMax=[]  IParamMin=[]  IParamMax=[]  DParamMin=[]  DParamMax=[]  NParamMin=[]  NParamMax=[]  KbParamMin=[]  KbParamMax=[]  KtParamMin=[]  KtParamMax=[]  KbOutMin=[]  KbOutMax=[]  KtOutMin=[]  KtOutMax=[]  IntegratorOutMin=[]  IntegratorOutMax=[]  FilterOutMin=[]  FilterOutMax=[]  SumI1OutMin=[]  SumI1OutMax=[]  SumI2OutMin=[]  SumI2OutMax=[]  SumI3OutMin=[]  SumI3OutMax=[]  SumI4OutMin=[]  SumI4OutMax=[]  SumDOutMin=[]  SumDOutMax=[]  DifferentiatorOutMin=[]  DifferentiatorOutMax=[]  FilterDiffOutCoefMin=[]  FilterDiffOutCoefMax=[]  ReciprocalOutMin=[]  ReciprocalOutMax=[]  SumDenOutMin=[]  SumDenOutMax=[]  SumNumOutMin=[]  SumNumOutMax=[]  DivideOutMin=[]  DivideOutMax=[]  UdiffTsProdOutMin=[]  UdiffTsProdOutMax=[]  NTsProdOutMin=[]  NTsProdOutMax=[]  UintegralTsProdOutMin=[]  UintegralTsProdOutMax=[]  UngainTsProdOutMin=[]  UngainTsProdOutMax=[]  ClampingZeroOutDataTypeStr=Inherit: Inherit via back propagation  ClampingZeroOutMin=[]  ClampingZeroOutMax=[]  FilterDenConstantOutDataTypeStr=Inherit: Inherit via back propagation  FilterDenConstantOutMin=[]  FilterDenConstantOutMax=[]  PCopyOutDataTypeStr=Inherit: Inherit via back propagation  PCopyOutMin=[]  PCopyOutMax=[]  NCopyOutDataTypeStr=Inherit: Inherit via back propagation  NCopyOutMin=[]  NCopyOutMax=[]  IntegratorContinuousStateAttributes=''  IntegratorStateMustResolveToSignalObject=off  IntegratorRTWStateStorageClass=Auto  FilterContinuousStateAttributes=''  FilterStateMustResolveToSignalObject=off  FilterRTWStateStorageClass=Auto  ParallelPVariant=InternalParameters  IdealPVariant=Disabled  IVariant=InternalParameters  DVariant=InternalParameters  IntegratorVariant=Continuous  SatVariant=Enabled  AWVariant=ContClampingParallel  PCopyVariant=Disabled  TRVariant=Disabled  FdbkBlocksVariant=Forward  IdealPFdbkVariant=Disabled  SatFdbkVariant=Disabled  DerivativeFilterVariant=ContFilter  NVariant=InternalParameters  NCopyVariant=Disabled  FilterICVariant=InternalICsFilter  IntegratorICVariant=InternalICs  ExternalResetVariant=Disabled  TRSumVariant=Passthrough  SumFdbkVariant=Disabled  SumVariant=Sum_PID  TsampFilterVariant=InternalTs  TsampNgainVariant=Passthrough  TsampIntegralVariant=Disabled_SignalSpec  ExternalSaturationOutDataTypeStr=Inherit: Same as second input  DerivativeSourceVariant=ErrorSignal  PreIntVariant=InternalPreInt
  Product{,1..5} (6 alike) : Product  Inputs=*/
  Selector : Selector  InputPortWidth=3  IndexOptions=Index vector (dialog)  Indices=3  OutputSizes=1
  Sum{,1,3,5..7} (6 alike) : Sum  Inputs=|+-
  Sum2 : Sum  Inputs=|++
  Sum4 : Sum  Inputs=|++
  Switch : Switch  Criteria=u2 > Threshold  SaturateOnIntegerOverflow=off  InputSameDT=off
  Unary Minus : UnaryMinus
  Theta_d : Outport
  Throttle : Outport  Port=2
  wires:
  Selector/1 -> Unary Minus/1
  Unary Minus/1 -> Sum/2  "h"
  Xe/1 -> Selector/1
  Sum/1 -> PID Controller/1
  h_d/1 -> Sum/1  "h_d"
  Airspeed/1 -> Derivative/1, MATLAB Function/1(Airspeed), Sum1/2
  Sum1/1 -> PID Controller1/1
  Derivative/1 -> [V_dot]
  gamma/1 -> [gamma]
  [V_dot_d] -> Product/1
  Constant/1 -> Product/2
  [h_dot_d] -> Product1/1
  [V] -> Product1/2
  Product/1 -> Sum2/1
  Product1/1 -> Sum2/2  "gamma_d"
  Sum2/1 -> Sum3/1  "E_dot_d"
  Product2/1 -> Sum4/1
  [V_dot] -> Product2/1
  Constant1/1 -> Product2/2
  [gamma] -> Sum4/2  "gamma"
  Sum4/1 -> Sum3/2  "E_dot"
  PID Controller3/1 -> Throttle/1
  [V] -> Product4/2
  [h_dot_d] -> Product4/1  "h_dot_d"
  Constant2/1 -> Product3/2
  [V_dot_d] -> Product3/1
  Product4/1 -> Sum5/1  "gamma_d"
  Product3/1 -> Sum5/2
  Sum5/1 -> Sum6/1  "B_dot_d"
  Constant3/1 -> Product5/2
  [V_dot] -> Product5/1
  [gamma] -> Sum7/1
  Product5/1 -> Sum7/2
  Sum7/1 -> Sum6/2  "B_dot"
  MATLAB Function/1(V) -> [V]
  PID Controller/1 -> [h_dot_d]
  PID Controller1/1 -> [V_dot_d]  "V_dot_d"
  Sum6/1 -> PID Controller2/1
  Sum3/1 -> PID Controller3/1
  PID Controller2/1 -> Theta_d/1
  Switch/1 -> Sum1/1  "Airspeed_d"
  Manual/1 -> Switch/2
  V_ref/1 -> Switch/3
  Airspeed_d/1 -> Switch/1

== system Y3Tiltrotor_sim3_INDI/Subsystem/固定翼模态/高度-速度控制/定速模式/airspeed control ==
  Manual : Inport
  Airspeed_d : Inport  Port=2
  V_ref : Inport  Port=3
  Airspeed : Inport  Port=4
  PID Controller1 : slpidlib/PID Controller  Controller=PID  Form=Parallel  TimeDomain=Continuous-time  UseExternalTs=off  SampleTime=ControlSampleTime  IntegratorMethod=Forward Euler  FilterMethod=Forward Euler  ControllerParametersSource=internal  P=control.FW.airspeed_P  I=control.FW.airspeed_I  UseKiTs=off  D=control.FW.airspeed_D  UseExternalDerivativeSource=off  N=100  UseFilter=on  TunerSelectOption=Transfer Function Based (PID Tuner App)  InitialConditionSource=internal  InitialConditionForIntegrator=0  InitialConditionForFilter=0  DifferentiatorICPrevScaledInput=0  ExternalReset=none  TrackingMode=off  Kt=1  LimitOutput=on  SatLimitsSource=internal  UpperSaturationLimit=1  LowerSaturationLimit=0  LinearizeAsGain=on  AntiWindupMode=clamping  Kb=1  LimitIntegrator=off  UpperIntegratorSaturationLimit=inf  LowerIntegratorSaturationLimit=-inf  POutMin=[]  POutMax=[]  IOutMin=[]  IOutMax=[]  DOutMin=[]  DOutMax=[]  NOutMin=[]  NOutMax=[]  SumOutMin=[]  SumOutMax=[]  SaturationOutMin=[]  SaturationOutMax=[]  PParamMin=[]  PParamMax=[]  IParamMin=[]  IParamMax=[]  DParamMin=[]  DParamMax=[]  NParamMin=[]  NParamMax=[]  KbParamMin=[]  KbParamMax=[]  KtParamMin=[]  KtParamMax=[]  KbOutMin=[]  KbOutMax=[]  KtOutMin=[]  KtOutMax=[]  IntegratorOutMin=[]  IntegratorOutMax=[]  FilterOutMin=[]  FilterOutMax=[]  SumI1OutMin=[]  SumI1OutMax=[]  SumI2OutMin=[]  SumI2OutMax=[]  SumI3OutMin=[]  SumI3OutMax=[]  SumI4OutMin=[]  SumI4OutMax=[]  SumDOutMin=[]  SumDOutMax=[]  DifferentiatorOutMin=[]  DifferentiatorOutMax=[]  FilterDiffOutCoefMin=[]  FilterDiffOutCoefMax=[]  ReciprocalOutMin=[]  ReciprocalOutMax=[]  SumDenOutMin=[]  SumDenOutMax=[]  SumNumOutMin=[]  SumNumOutMax=[]  DivideOutMin=[]  DivideOutMax=[]  UdiffTsProdOutMin=[]  UdiffTsProdOutMax=[]  NTsProdOutMin=[]  NTsProdOutMax=[]  UintegralTsProdOutMin=[]  UintegralTsProdOutMax=[]  UngainTsProdOutMin=[]  UngainTsProdOutMax=[]  ClampingZeroOutDataTypeStr=Inherit: Inherit via back propagation  ClampingZeroOutMin=[]  ClampingZeroOutMax=[]  FilterDenConstantOutDataTypeStr=Inherit: Inherit via back propagation  FilterDenConstantOutMin=[]  FilterDenConstantOutMax=[]  PCopyOutDataTypeStr=Inherit: Inherit via back propagation  PCopyOutMin=[]  PCopyOutMax=[]  NCopyOutDataTypeStr=Inherit: Inherit via back propagation  NCopyOutMin=[]  NCopyOutMax=[]  IntegratorContinuousStateAttributes=''  IntegratorStateMustResolveToSignalObject=off  IntegratorRTWStateStorageClass=Auto  FilterContinuousStateAttributes=''  FilterStateMustResolveToSignalObject=off  FilterRTWStateStorageClass=Auto  ParallelPVariant=InternalParameters  IdealPVariant=Disabled  IVariant=InternalParameters  DVariant=InternalParameters  IntegratorVariant=Continuous  SatVariant=Enabled  AWVariant=ContClampingParallel  PCopyVariant=Disabled  TRVariant=Disabled  FdbkBlocksVariant=Forward  IdealPFdbkVariant=Disabled  SatFdbkVariant=Disabled  DerivativeFilterVariant=ContFilter  NVariant=InternalParameters  NCopyVariant=Disabled  FilterICVariant=InternalICsFilter  IntegratorICVariant=InternalICs  ExternalResetVariant=Disabled  TRSumVariant=Passthrough  SumFdbkVariant=Disabled  SumVariant=Sum_PID  TsampFilterVariant=InternalTs  TsampNgainVariant=Passthrough  TsampIntegralVariant=Disabled_SignalSpec  ExternalSaturationOutDataTypeStr=Inherit: Same as second input  DerivativeSourceVariant=ErrorSignal  PreIntVariant=InternalPreInt
  Sum : Sum  Inputs=|+-
  Switch : Switch  Criteria=u2 > Threshold  SaturateOnIntegerOverflow=off  InputSameDT=off
  Throttle : Outport
  wires:
  Sum/1 -> PID Controller1/1
  Airspeed/1 -> Sum/2
  PID Controller1/1 -> Throttle/1
  Switch/1 -> Sum/1
  Manual/1 -> Switch/2
  Airspeed_d/1 -> Switch/1
  V_ref/1 -> Switch/3

== system Y3Tiltrotor_sim3_INDI/Subsystem/固定翼模态/高度-速度控制/定高模式/Subsystem ==
  Manual : Inport
  Height_d : Inport  Port=2
  Manual Vz_d : Inport  Port=3
  Xe : Inport  Port=4
  InputConditioning_altitude : Subsystem
  Merge : Merge
  Subsystem : Subsystem
  Switch Case : SwitchCase  CaseConditions={0,1}  ShowDefaultCase=off
  Vz_d : Outport
  wires:
  Manual/1 -> Switch Case/1
  Xe/1 -> Subsystem/2(Xe), InputConditioning_altitude/2(Xe)
  Subsystem/1(PID_vz_cmd) -> Merge/1  "PID vz_d"
  InputConditioning_altitude/1(manual_vz_cmd) -> Merge/2  "Manual vz_d"
  Merge/1 -> Vz_d/1
  Switch Case/1 -> Subsystem/Action
  Switch Case/2 -> InputConditioning_altitude/Action
  Manual Vz_d/1 -> InputConditioning_altitude/1(Manual Vz_d)
  Height_d/1 -> Subsystem/1(Navigation Z)

== system Y3Tiltrotor_sim3_INDI/Subsystem/多旋翼模态/Multirotor XY control/Subsystem/InputConditioning_altitude ==
  Ch2 : Inport
  Action Port : ActionPort  ActionPortLabel=case [ 1 ]:
  Saturation1 : Saturate  UpperLimit=1  LowerLimit=-1
  deadzone3 : MATLAB Function  TreatAsAtomicUnit=on
  max_vy : Gain  Gain=control.maxMRvelocity_lat  OutDataTypeStr=Inherit: Inherit via back propagation
  manual_vlat_cmd : Outport  VectorParamsAs1DForOutWhenUnconnected=off
  wires:
  Ch2/1 -> deadzone3/1(u)
  deadzone3/1(y) -> Saturation1/1
  Saturation1/1 -> max_vy/1
  max_vy/1 -> manual_vlat_cmd/1
